simulink model "pid_analog_circuit"  (R2024b)
settings: Solver=ode4  StartTime=0.0  StopTime=1  FixedStep=pcb.sim_dt  RelTol=1e-3
PostLoadFcn:
  | pacdir_ = fileparts(get_param('pid_analog_circuit','FileName')); if ~exist('pcb','var'), run(fullfile(pacdir_,'pid_board_params.m')); end; if ~exist('pacirc','var'), run(fullfile(pacdir_,'pid_analog_circuit_params.m')); end; clear pacdir_
values from neighbouring files (symbols this model uses):
  pacirc = struct()    [pid_analog_circuit_params.m]
  pcb = evalin('base', 'pcb')    [pid_analog_circuit_test.m]    (also in pid_board_bench_inputs.m; pid_board_params.m = struct(); pid_board_validate.m)
libraries: ee_lib x153, fl_lib x61, nesl_utility x48
(part 3 of 5)

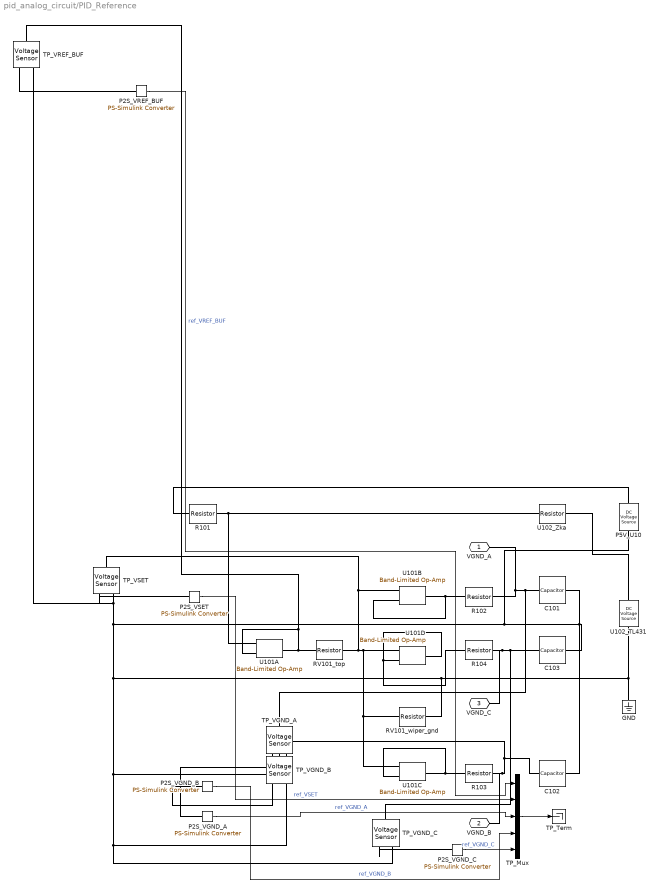
== system pid_analog_circuit/PID_Reference ==
  C101 : ee_lib/Passive/Capacitor  cap_option=ee.enum.passive.capacitor.capOption.const  c=pcb.ref.C_rail F  Cvec=[1e-05, 1e-06] F  Vvec=[0, 10] V  CV_table_symmetry=ee.enum.passive.capacitor.tableSymmetry.yes  f_vec=[1, 10] kHz  DFext_vec=[.8, 1.2]  enable_C_tol=ee.enum.toleranceApplication.none  averaging_period=0 s  C_tol=5  tol_distribution=ee.enum.toleranceDistribution.uniform  nSigma=4  r=0 Ohm  g=0 1/Ohm  enable_operating_limits=ee.enum.enable.no  operating_limit_action=ee.enum.passive.reportOpLim.warn  max_working_voltage_range=[-25, 25] V  power_rating=1 W  maxTemperature=85 degC  thermalEnable=false  thermalMass=1 J/K  fault_action=simscape.enum.assert.action.none  t_fault=1 s  i_specify=off  i_priority=None  i=0 A  i_nominal_specify=off  i_nominal_value=1  i_nominal_unit=A  v_specify=off  v_priority=None  v=0 V  v_nominal_specify=off  v_nominal_value=1  v_nominal_unit=V  vc_specify=on  vc_priority=High  vc=pacirc.V0_rail V  vc_nominal_specify=off  vc_nominal_value=1  vc_nominal_unit=V  T_specify=off  T_priority=None  T=298.15 K  T_nominal_specify=off  T_nominal_value=1  T_nominal_unit=K
  C102 : ee_lib/Passive/Capacitor  cap_option=ee.enum.passive.capacitor.capOption.const  c=pcb.ref.C_rail F  Cvec=[1e-05, 1e-06] F  Vvec=[0, 10] V  CV_table_symmetry=ee.enum.passive.capacitor.tableSymmetry.yes  f_vec=[1, 10] kHz  DFext_vec=[.8, 1.2]  enable_C_tol=ee.enum.toleranceApplication.none  averaging_period=0 s  C_tol=5  tol_distribution=ee.enum.toleranceDistribution.uniform  nSigma=4  r=0 Ohm  g=0 1/Ohm  enable_operating_limits=ee.enum.enable.no  operating_limit_action=ee.enum.passive.reportOpLim.warn  max_working_voltage_range=[-25, 25] V  power_rating=1 W  maxTemperature=85 degC  thermalEnable=false  thermalMass=1 J/K  fault_action=simscape.enum.assert.action.none  t_fault=1 s  i_specify=off  i_priority=None  i=0 A  i_nominal_specify=off  i_nominal_value=1  i_nominal_unit=A  v_specify=off  v_priority=None  v=0 V  v_nominal_specify=off  v_nominal_value=1  v_nominal_unit=V  vc_specify=on  vc_priority=High  vc=pacirc.V0_rail V  vc_nominal_specify=off  vc_nominal_value=1  vc_nominal_unit=V  T_specify=off  T_priority=None  T=298.15 K  T_nominal_specify=off  T_nominal_value=1  T_nominal_unit=K
  C103 : ee_lib/Passive/Capacitor  cap_option=ee.enum.passive.capacitor.capOption.const  c=pcb.ref.C_rail F  Cvec=[1e-05, 1e-06] F  Vvec=[0, 10] V  CV_table_symmetry=ee.enum.passive.capacitor.tableSymmetry.yes  f_vec=[1, 10] kHz  DFext_vec=[.8, 1.2]  enable_C_tol=ee.enum.toleranceApplication.none  averaging_period=0 s  C_tol=5  tol_distribution=ee.enum.toleranceDistribution.uniform  nSigma=4  r=0 Ohm  g=0 1/Ohm  enable_operating_limits=ee.enum.enable.no  operating_limit_action=ee.enum.passive.reportOpLim.warn  max_working_voltage_range=[-25, 25] V  power_rating=1 W  maxTemperature=85 degC  thermalEnable=false  thermalMass=1 J/K  fault_action=simscape.enum.assert.action.none  t_fault=1 s  i_specify=off  i_priority=None  i=0 A  i_nominal_specify=off  i_nominal_value=1  i_nominal_unit=A  v_specify=off  v_priority=None  v=0 V  v_nominal_specify=off  v_nominal_value=1  v_nominal_unit=V  vc_specify=on  vc_priority=High  vc=pacirc.V0_rail V  vc_nominal_specify=off  vc_nominal_value=1  vc_nominal_unit=V  T_specify=off  T_priority=None  T=298.15 K  T_nominal_specify=off  T_nominal_value=1  T_nominal_unit=K
  GND : fl_lib/Electrical/Electrical Elements/Electrical Reference
  P2S_VGND_A : nesl_utility/PS-Simulink Converter  PhysicalDomain=network_engine_domain  SubClassName=ps_output  LeftPortType=input  RightPortType=output  PseudoPeriodic=off  Frequencies=[]  VectorFormat=inherit  Unit=V  AffineConversion=off
  P2S_VGND_B : nesl_utility/PS-Simulink Converter  PhysicalDomain=network_engine_domain  SubClassName=ps_output  LeftPortType=input  RightPortType=output  PseudoPeriodic=off  Frequencies=[]  VectorFormat=inherit  Unit=V  AffineConversion=off
  P2S_VGND_C : nesl_utility/PS-Simulink Converter  PhysicalDomain=network_engine_domain  SubClassName=ps_output  LeftPortType=input  RightPortType=output  PseudoPeriodic=off  Frequencies=[]  VectorFormat=inherit  Unit=V  AffineConversion=off
  P2S_VREF_BUF : nesl_utility/PS-Simulink Converter  PhysicalDomain=network_engine_domain  SubClassName=ps_output  LeftPortType=input  RightPortType=output  PseudoPeriodic=off  Frequencies=[]  VectorFormat=inherit  Unit=V  AffineConversion=off
  P2S_VSET : nesl_utility/PS-Simulink Converter  PhysicalDomain=network_engine_domain  SubClassName=ps_output  LeftPortType=input  RightPortType=output  PseudoPeriodic=off  Frequencies=[]  VectorFormat=inherit  Unit=V  AffineConversion=off
  P5V_U10 : fl_lib/Electrical/Electrical Sources/DC Voltage Source  v0=pcb.VDD V
  R101 : ee_lib/Passive/Resistor  R=pcb.ref.R_bias Ohm  enable_R_tol=ee.enum.toleranceApplication.none  R_tol=5  tol_distribution=ee.enum.toleranceDistribution.uniform  nSigma=4  enable_operating_limits=ee.enum.enable.no  operating_limit_action=ee.enum.passive.reportOpLim.warn  power_rating=1 W  max_working_voltage=100 V  noise_mode=ee.enum.sources.noise.Disabled  Tdevice=25 degC  sample_time=1e-3 s  repeatability=ee.enum.ic.repeatability.notRepeatable  user_seed=0  auto_seed=3237241810  fault_action=simscape.enum.assert.action.none  t_fault=1 s  power_derating_T1=70 degC  power_derating_T2=155 degC  operating_temperature_range_vec=[-50, 150] degC  alpha=3.93e-3 1/K  Tmeas=25 degC  thermal_mass=100 J/K  temperature_specify=off  temperature_priority=High  temperature=298.15 K  temperature_nominal_specify=off  temperature_nominal_value=1  temperature_nominal_unit=K
  R102 : ee_lib/Passive/Resistor  R=pcb.ref.R_iso Ohm  enable_R_tol=ee.enum.toleranceApplication.none  R_tol=5  tol_distribution=ee.enum.toleranceDistribution.uniform  nSigma=4  enable_operating_limits=ee.enum.enable.no  operating_limit_action=ee.enum.passive.reportOpLim.warn  power_rating=1 W  max_working_voltage=100 V  noise_mode=ee.enum.sources.noise.Disabled  Tdevice=25 degC  sample_time=1e-3 s  repeatability=ee.enum.ic.repeatability.notRepeatable  user_seed=0  auto_seed=231713996  fault_action=simscape.enum.assert.action.none  t_fault=1 s  power_derating_T1=70 degC  power_derating_T2=155 degC  operating_temperature_range_vec=[-50, 150] degC  alpha=3.93e-3 1/K  Tmeas=25 degC  thermal_mass=100 J/K  temperature_specify=off  temperature_priority=High  temperature=298.15 K  temperature_nominal_specify=off  temperature_nominal_value=1  temperature_nominal_unit=K
  R103 : ee_lib/Passive/Resistor  R=pcb.ref.R_iso Ohm  enable_R_tol=ee.enum.toleranceApplication.none  R_tol=5  tol_distribution=ee.enum.toleranceDistribution.uniform  nSigma=4  enable_operating_limits=ee.enum.enable.no  operating_limit_action=ee.enum.passive.reportOpLim.warn  power_rating=1 W  max_working_voltage=100 V  noise_mode=ee.enum.sources.noise.Disabled  Tdevice=25 degC  sample_time=1e-3 s  repeatability=ee.enum.ic.repeatability.notRepeatable  user_seed=0  auto_seed=2279758131  fault_action=simscape.enum.assert.action.none  t_fault=1 s  power_derating_T1=70 degC  power_derating_T2=155 degC  operating_temperature_range_vec=[-50, 150] degC  alpha=3.93e-3 1/K  Tmeas=25 degC  thermal_mass=100 J/K  temperature_specify=off  temperature_priority=High  temperature=298.15 K  temperature_nominal_specify=off  temperature_nominal_value=1  temperature_nominal_unit=K
  R104 : ee_lib/Passive/Resistor  R=pcb.ref.R_iso Ohm  enable_R_tol=ee.enum.toleranceApplication.none  R_tol=5  tol_distribution=ee.enum.toleranceDistribution.uniform  nSigma=4  enable_operating_limits=ee.enum.enable.no  operating_limit_action=ee.enum.passive.reportOpLim.warn  power_rating=1 W  max_working_voltage=100 V  noise_mode=ee.enum.sources.noise.Disabled  Tdevice=25 degC  sample_time=1e-3 s  repeatability=ee.enum.ic.repeatability.notRepeatable  user_seed=0  auto_seed=3346497771  fault_action=simscape.enum.assert.action.none  t_fault=1 s  power_derating_T1=70 degC  power_derating_T2=155 degC  operating_temperature_range_vec=[-50, 150] degC  alpha=3.93e-3 1/K  Tmeas=25 degC  thermal_mass=100 J/K  temperature_specify=off  temperature_priority=High  temperature=298.15 K  temperature_nominal_specify=off  temperature_nominal_value=1  temperature_nominal_unit=K
  RV101_top : ee_lib/Passive/Resistor  R=max(pcb.ref.RV_set - pacirc.ref.RV_wg, 1e-3) Ohm  enable_R_tol=ee.enum.toleranceApplication.none  R_tol=5  tol_distribution=ee.enum.toleranceDistribution.uniform  nSigma=4  enable_operating_limits=ee.enum.enable.no  operating_limit_action=ee.enum.passive.reportOpLim.warn  power_rating=1 W  max_working_voltage=100 V  noise_mode=ee.enum.sources.noise.Disabled  Tdevice=25 degC  sample_time=1e-3 s  repeatability=ee.enum.ic.repeatability.notRepeatable  user_seed=0  auto_seed=2438775377  fault_action=simscape.enum.assert.action.none  t_fault=1 s  power_derating_T1=70 degC  power_derating_T2=155 degC  operating_temperature_range_vec=[-50, 150] degC  alpha=3.93e-3 1/K  Tmeas=25 degC  thermal_mass=100 J/K  temperature_specify=off  temperature_priority=High  temperature=298.15 K  temperature_nominal_specify=off  temperature_nominal_value=1  temperature_nominal_unit=K
  RV101_wiper_gnd : ee_lib/Passive/Resistor  R=max(pacirc.ref.RV_wg, 1e-3) Ohm  enable_R_tol=ee.enum.toleranceApplication.none  R_tol=5  tol_distribution=ee.enum.toleranceDistribution.uniform  nSigma=4  enable_operating_limits=ee.enum.enable.no  operating_limit_action=ee.enum.passive.reportOpLim.warn  power_rating=1 W  max_working_voltage=100 V  noise_mode=ee.enum.sources.noise.Disabled  Tdevice=25 degC  sample_time=1e-3 s  repeatability=ee.enum.ic.repeatability.notRepeatable  user_seed=0  auto_seed=325791693  fault_action=simscape.enum.assert.action.none  t_fault=1 s  power_derating_T1=70 degC  power_derating_T2=155 degC  operating_temperature_range_vec=[-50, 150] degC  alpha=3.93e-3 1/K  Tmeas=25 degC  thermal_mass=100 J/K  temperature_specify=off  temperature_priority=High  temperature=298.15 K  temperature_nominal_specify=off  temperature_nominal_value=1  temperature_nominal_unit=K
  TP_Mux : Mux  Inputs=5
  TP_Term : Terminator
  TP_VGND_A : fl_lib/Electrical/Electrical Sensors/Voltage Sensor
  TP_VGND_B : fl_lib/Electrical/Electrical Sensors/Voltage Sensor
  TP_VGND_C : fl_lib/Electrical/Electrical Sensors/Voltage Sensor
  TP_VREF_BUF : fl_lib/Electrical/Electrical Sensors/Voltage Sensor
  TP_VSET : fl_lib/Electrical/Electrical Sensors/Voltage Sensor
  U101A : ee_lib/Integrated Circuits/Band-Limited Op-Amp  A=pacirc.opamp.A  Rin=pacirc.opamp.Rin Ohm  Rout=pacirc.opamp.Rout Ohm  Vmin=pacirc.opamp.Vmin V  Vmax=pacirc.opamp.Vmax V  Vdotmax=pacirc.opamp.SR V/s  f=pacirc.opamp.f Hz  V0=pcb.ref.V_tl431 V
  U101B : ee_lib/Integrated Circuits/Band-Limited Op-Amp  A=pacirc.opamp.A  Rin=pacirc.opamp.Rin Ohm  Rout=pacirc.opamp.Rout Ohm  Vmin=pacirc.opamp.Vmin V  Vmax=pacirc.opamp.Vmax V  Vdotmax=pacirc.opamp.SR V/s  f=pacirc.opamp.f Hz  V0=pacirc.opamp.V0 V
  U101C : ee_lib/Integrated Circuits/Band-Limited Op-Amp  A=pacirc.opamp.A  Rin=pacirc.opamp.Rin Ohm  Rout=pacirc.opamp.Rout Ohm  Vmin=pacirc.opamp.Vmin V  Vmax=pacirc.opamp.Vmax V  Vdotmax=pacirc.opamp.SR V/s  f=pacirc.opamp.f Hz  V0=pacirc.opamp.V0 V
  U101D : ee_lib/Integrated Circuits/Band-Limited Op-Amp  A=pacirc.opamp.A  Rin=pacirc.opamp.Rin Ohm  Rout=pacirc.opamp.Rout Ohm  Vmin=pacirc.opamp.Vmin V  Vmax=pacirc.opamp.Vmax V  Vdotmax=pacirc.opamp.SR V/s  f=pacirc.opamp.f Hz  V0=pacirc.opamp.V0 V
  U102_TL431 : fl_lib/Electrical/Electrical Sources/DC Voltage Source  v0=pcb.ref.V_tl431 V
  U102_Zka : ee_lib/Passive/Resistor  R=pacirc.ref.R_tl431 Ohm  enable_R_tol=ee.enum.toleranceApplication.none  R_tol=5  tol_distribution=ee.enum.toleranceDistribution.uniform  nSigma=4  enable_operating_limits=ee.enum.enable.no  operating_limit_action=ee.enum.passive.reportOpLim.warn  power_rating=1 W  max_working_voltage=100 V  noise_mode=ee.enum.sources.noise.Disabled  Tdevice=25 degC  sample_time=1e-3 s  repeatability=ee.enum.ic.repeatability.notRepeatable  user_seed=0  auto_seed=1634002471  fault_action=simscape.enum.assert.action.none  t_fault=1 s  power_derating_T1=70 degC  power_derating_T2=155 degC  operating_temperature_range_vec=[-50, 150] degC  alpha=3.93e-3 1/K  Tmeas=25 degC  thermal_mass=100 J/K  temperature_specify=off  temperature_priority=High  temperature=298.15 K  temperature_nominal_specify=off  temperature_nominal_value=1  temperature_nominal_unit=K
  VGND_A : PMIOPort  Side=Right
  VGND_B : PMIOPort  Port=2  Side=Right
  VGND_C : PMIOPort  Port=3  Side=Right
  wires:
  P2S_VGND_C/1 -> TP_Mux/5  "ref_VGND_C"
  P2S_VGND_B/1 -> TP_Mux/4  "ref_VGND_B"
  P2S_VGND_A/1 -> TP_Mux/3  "ref_VGND_A"
  P2S_VSET/1 -> TP_Mux/2  "ref_VSET"
  P2S_VREF_BUF/1 -> TP_Mux/1  "ref_VREF_BUF"
  TP_Mux/1 -> TP_Term/1
  connections:
  C102/LConn1 -- R103/RConn1 -- VGND_B/RConn1 -- TP_VGND_B/LConn1
  VGND_A/RConn1 -- C101/LConn1 -- TP_VGND_A/LConn1 -- R102/RConn1
  R104/LConn1 -- U101D/LConn2 -- U101D/RConn1
  U101C/RConn1 -- R103/LConn1 -- U101C/LConn2
  U101B/RConn1 -- R102/LConn1 -- U101B/LConn2
  U102_Zka/RConn1 -- U102_TL431/LConn1
  R101/RConn1 -- U101A/LConn1 -- U102_Zka/LConn1
  P5V_U10/LConn1 -- R101/LConn1
  C103/RConn1 -- TP_VGND_C/RConn2 -- TP_VGND_B/RConn2 -- TP_VGND_A/RConn2 -- GND/LConn1 -- U102_TL431/RConn1 -- RV101_wiper_gnd/RConn1 -- TP_VSET/RConn2 -- TP_VREF_BUF/RConn2 -- P5V_U10/RConn1 -- C102/RConn1 -- C101/RConn1
  U101A/LConn2 -- U101A/RConn1 -- RV101_top/LConn1 -- TP_VREF_BUF/LConn1
  U101C/LConn1 -- RV101_top/RConn1 -- U101B/LConn1 -- TP_VSET/LConn1 -- U101D/LConn1 -- RV101_wiper_gnd/LConn1
  C103/LConn1 -- R104/RConn1 -- VGND_C/RConn1 -- TP_VGND_C/LConn1
  TP_VGND_C/RConn1 -- P2S_VGND_C/LConn1
  TP_VGND_B/RConn1 -- P2S_VGND_B/LConn1
  TP_VGND_A/RConn1 -- P2S_VGND_A/LConn1
  TP_VSET/RConn1 -- P2S_VSET/LConn1
  TP_VREF_BUF/RConn1 -- P2S_VREF_BUF/LConn1
